simulink model "mimo_test6"  (R2025b)
settings: Solver=ode8  StartTime=0.0  StopTime=10.0  FixedStep=0.01  RelTol=1e-3
settings Model: Creator=MehrSystem  LastModifiedBy=MehrSystem

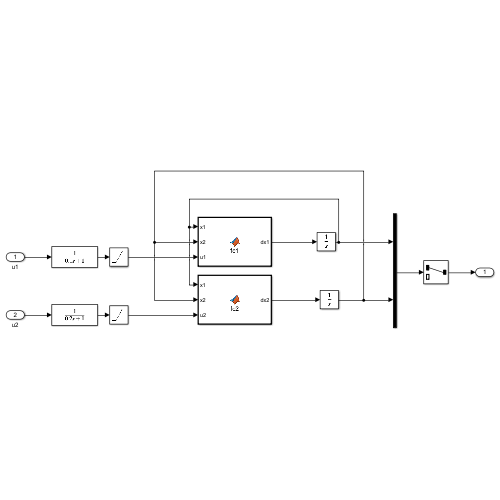
[thumbnail: Simulink's stored preview of the top-level diagram]
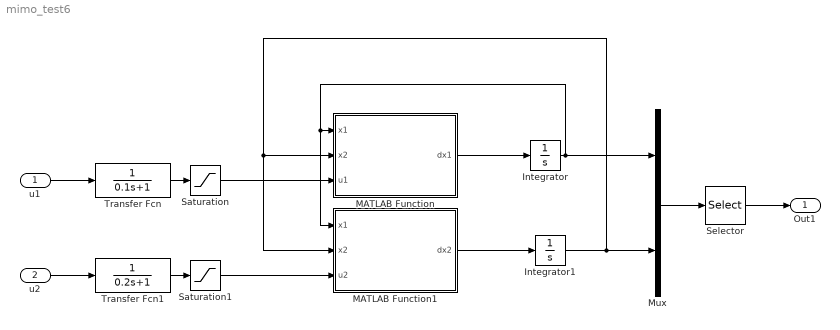
== system mimo_test6 ==
  u1 : Inport
  u2 : Inport  Port=2
  Integrator : Integrator
  Integrator1 : Integrator
  MATLAB Function : MATLAB Function  TreatAsAtomicUnit=on
  MATLAB Function1 : MATLAB Function  TreatAsAtomicUnit=on
  Mux : Mux  Inputs=2
  Saturation : Saturate  UpperLimit=0.7  LowerLimit=-0.9
  Saturation1 : Saturate  UpperLimit=0.95  LowerLimit=-0.85
  Selector : Selector  InputPortWidth=2  IndexOptions=Index vector (dialog)  Indices=[1]  OutputSizes=1
  Transfer Fcn : TransferFcn  Denominator=[0.1 1]
  Transfer Fcn1 : TransferFcn  Denominator=[0.2 1]
  Out1 : Outport
  wires:
  MATLAB Function/1(dx1) -> Integrator/1
  MATLAB Function1/1(dx2) -> Integrator1/1
  u1/1 -> Transfer Fcn/1
  u2/1 -> Transfer Fcn1/1
  Saturation/1 -> MATLAB Function/3(u1)
  Saturation1/1 -> MATLAB Function1/3(u2)
  Integrator/1 -> MATLAB Function1/1(x1), MATLAB Function/1(x1), Mux/1
  Integrator1/1 -> MATLAB Function/2(x2), MATLAB Function1/2(x2), Mux/2
  Mux/1 -> Selector/1
  Selector/1 -> Out1/1
  Transfer Fcn/1 -> Saturation/1
  Transfer Fcn1/1 -> Saturation1/1

== matlab function mimo_test6/MATLAB Function ==
  data: x1 input; dx1 output; x2 input; u1 input
function dx1 = fc1(x1, x2, u1)
    % State 1 dynamics

    a11 = -0.5;
    a12 = 0.2;
    b1  = 1.0;

    dx1 = a11 * x1 + a12 * x2 + b1 * u1;
end

== matlab function mimo_test6/MATLAB Function1 ==
  data: x1 input; dx2 output; x2 input; u2 input
function dx2 = fc2(x1, x2, u2)
    % State 2 dynamics

    a21 = 0.1;
    a22 = -0.3;
    b2  = 1.5;

    dx2 = a21 * x1 + a22 * x2 + b2 * u2;
end
